simulink model "IT_Independent_HeatRejection_20261023_SK"  (R2026a)
settings: Solver=FixedStepDiscrete  StopTime=3600  FixedStep=5
undefined symbols (not defined in the file or in its folder): safe_params
settings Model: Creator=Lysda  LastModifiedBy=Lysda

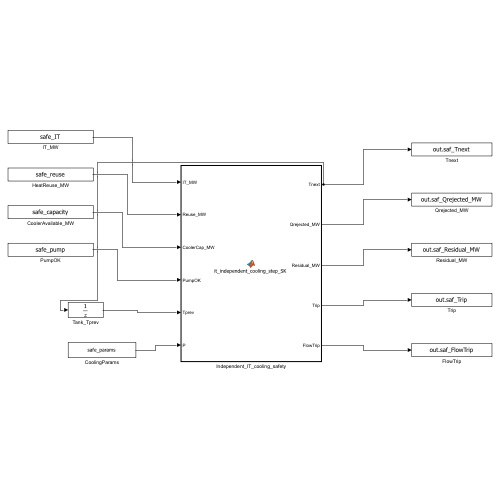
[thumbnail: Simulink's stored preview of the top-level diagram]
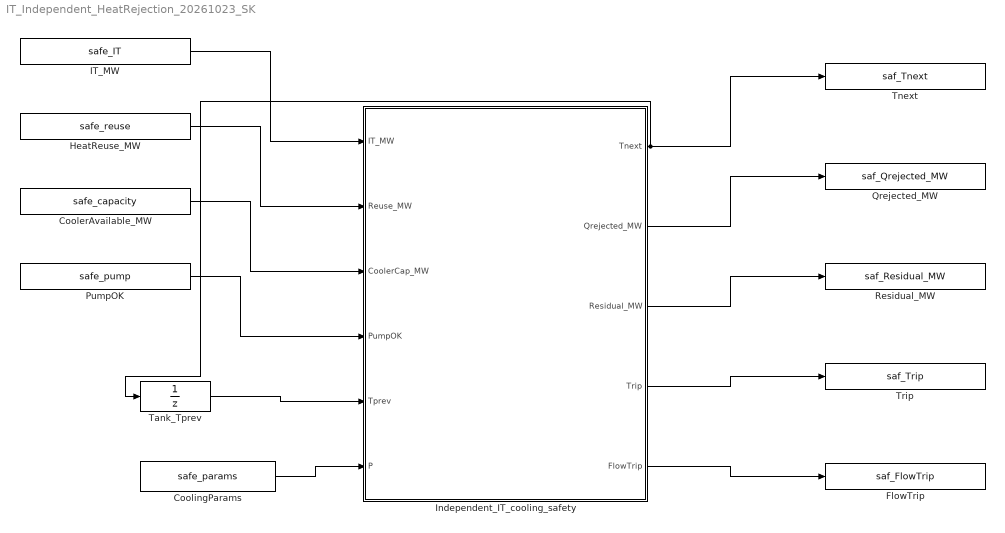
== system IT_Independent_HeatRejection_20261023_SK ==
  CoolerAvailable_MW : FromWorkspace  VariableName=safe_capacity
  CoolingParams : Constant  Value=safe_params
  FlowTrip : ToWorkspace  VariableName=saf_FlowTrip  SaveFormat=Timeseries  SampleTime=-1
  HeatReuse_MW : FromWorkspace  VariableName=safe_reuse
  IT_MW : FromWorkspace  VariableName=safe_IT
  Independent_IT_cooling_safety : MATLAB Function  TreatAsAtomicUnit=on
  PumpOK : FromWorkspace  VariableName=safe_pump
  Qrejected_MW : ToWorkspace  VariableName=saf_Qrejected_MW  SaveFormat=Timeseries  SampleTime=-1
  Residual_MW : ToWorkspace  VariableName=saf_Residual_MW  SaveFormat=Timeseries  SampleTime=-1
  Tank_Tprev : UnitDelay  InitialCondition=35  SampleTime=5
  Tnext : ToWorkspace  VariableName=saf_Tnext  SaveFormat=Timeseries  SampleTime=-1
  Trip : ToWorkspace  VariableName=saf_Trip  SaveFormat=Timeseries  SampleTime=-1
  wires:
  IT_MW/1 -> Independent_IT_cooling_safety/1(IT_MW)
  HeatReuse_MW/1 -> Independent_IT_cooling_safety/2(Reuse_MW)
  CoolerAvailable_MW/1 -> Independent_IT_cooling_safety/3(CoolerCap_MW)
  PumpOK/1 -> Independent_IT_cooling_safety/4(PumpOK)
  Tank_Tprev/1 -> Independent_IT_cooling_safety/5(Tprev)
  CoolingParams/1 -> Independent_IT_cooling_safety/6(P)
  Independent_IT_cooling_safety/1(Tnext) -> Tnext/1, Tank_Tprev/1
  Independent_IT_cooling_safety/2(Qrejected_MW) -> Qrejected_MW/1
  Independent_IT_cooling_safety/3(Residual_MW) -> Residual_MW/1
  Independent_IT_cooling_safety/4(Trip) -> Trip/1
  Independent_IT_cooling_safety/5(FlowTrip) -> FlowTrip/1

== matlab function IT_Independent_HeatRejection_20261023_SK/Independent_IT_cooling_safety ==
  data: IT_MW input; Tnext output; Reuse_MW input; CoolerCap_MW input; PumpOK input; Tprev input; P input; Qrejected_MW output; Residual_MW output; Trip output; FlowTrip output
function [Tnext,Qrejected_MW,Residual_MW,Trip,FlowTrip] = ...
 it_independent_cooling_step_SK(IT_MW,Reuse_MW,CoolerCap_MW,PumpOK,Tprev,P)
%#codegen
% IT safety thermal buffer, independent rejection capacity. Screening, not PLC.
% P = [rhoVcp_JK, dt_s, normal_T_C, max_T_C]
C=P(1);dt=P(2);Tnom=P(3);Tmax=P(4);
qIT=max(0,IT_MW);
use=max(0,min(qIT,Reuse_MW));
qtoReject=qIT-use;
FlowTrip=double(PumpOK<0.5);
if PumpOK>=0.5
  available=max(0,CoolerCap_MW);
  buffered=max(0,Tprev-Tnom)*C/(dt*1e6);
  Qrejected_MW=min(available,qtoReject+buffered);
else
  % Flow fault -> heat recovery and rejection cannot protect chips.
  Qrejected_MW=0;
  qtoReject=qIT;
end
Residual_MW=qtoReject-Qrejected_MW;
Tnext=Tprev+Residual_MW*1e6*dt/C;
Trip=double(Tnext>Tmax || FlowTrip>0.5);
end
